simulink model "inv_psm"  (R2026b)
settings: Solver=ode23tb  StopTime=param.sim.simlength  FixedStep=param.sim.tc  MaxStep=param.glb_time.tc
values from neighbouring files (symbols this model uses):
  param = struct()    [init_model.m]
undefined symbols (not defined in the file or in its folder): magnitude
libraries: fl_lib x155, nesl_utility x77, igbt_simple_2th_lib x6, lithium_ion_battery x2, simple_flexible_shaft x2, cstblocks_lti x2, dclink_with_center_tap x1, three_phase_pwm_modulator x1, three_phase_inverter_ideal_switch_based_model x1, three_phase_inverter_igbt_advanced_thermal_model x1, three_phase_inverter_mosfet_based_with_thermal_model x1, threephase_inductor_lib x1
(part 6 of 6)

== system inv_psm/inv_psm_mod1/inverter_ctrl/inverter_control/current_ctrl/current_ctrl/dq_pi_with_vector_antiwindup mod1/dq_vector_pi/vector lenght ==
  md : Inport
  mq : Inport  Port=2
  Math Function : Math  Operator=magnitude^2  SignedPower=on
  Math Function1 : Math  Operator=magnitude^2  SignedPower=on
  Math Function2 : Math  Operator=reciprocal  SignedPower=on
  Sqrt : Sqrt
  Sum5 : Sum  SaturateOnIntegerOverflow=on
  m_1 : Outport  VectorParamsAs1DForOutWhenUnconnected=off
  m : Outport  Port=2  VectorParamsAs1DForOutWhenUnconnected=off
  wires:
  Sqrt/1 -> m/1, Math Function2/1
  mq/1 -> Math Function1/1
  Math Function1/1 -> Sum5/2
  Math Function/1 -> Sum5/1
  Sum5/1 -> Sqrt/1
  Math Function2/1 -> m_1/1
  md/1 -> Math Function/1

== system inv_psm/inv_psm_mod1/inverter_ctrl/inverter_control/current_ctrl/current_ctrl/dq_pi_with_vector_antiwindup mod1/dq_vector_pi_ccaller/Reset ==
  Step : Step  Time=0.05  InitialValue=1  FinalValue=0
  en : Outport
  wires:
  Step/1 -> en/1

== system inv_psm/inv_psm_mod1/inverter_ctrl/inverter_control/current_ctrl/bemf_observer/EKF_bemf_observer/extended_kalman_observer/correlation_matrix/A_ekf ==
  Gain1 : Gain  Gain=param.psm.ctrl.ekf.A6_tilde_ekf
  Gain{7..10,13,20} (6 alike) : Gain  Gain=param.psm.machine.omega_bez
  Gain{2,4,6,11,16,18} (6 alike) : Gain  Gain=param.glb_time.ts_inv
  Gain15 : Gain  Gain=param.psm.ctrl.ekf.A2_tilde_ekf
  Gain17 : Gain  Gain=param.psm.ctrl.ekf.A3_tilde_ekf
  Gain3 : Gain  Gain=param.psm.ctrl.ekf.A4_tilde_ekf
  Gain5 : Gain  Gain=param.psm.ctrl.ekf.A5_tilde_ekf
  I1 : Constant  Value=eye(6)
  I2 : Constant  Value=param.psm.ctrl.ekf.A1_tilde_ekf
  Sum7 : Sum  Inputs=+++++++
  out : Outport
  wires:
  Sum7/1 -> out/1
  I2/1 -> Gain11/1
  I1/1 -> Sum7/1
  Gain1/1 -> Gain2/1
  Gain3/1 -> Gain4/1
  Gain5/1 -> Gain6/1
  [omega_hat_kalman] -> Gain1/1
  [psi_alpha_hat] -> Gain3/1
  [psi_beta_hat] -> Gain5/1
  Gain11/1 -> Gain7/1
  Gain2/1 -> Gain8/1
  Gain4/1 -> Gain9/1
  Gain6/1 -> Gain10/1
  Gain7/1 -> Sum7/2
  Gain9/1 -> Sum7/5
  Gain10/1 -> Sum7/6
  Gain8/1 -> Sum7/7
  Gain18/1 -> Gain13/1
  Gain16/1 -> Gain20/1
  Gain17/1 -> Gain18/1
  Gain15/1 -> Gain16/1
  Gain13/1 -> Sum7/4
  Gain20/1 -> Sum7/3
  [i_beta_hat] -> Gain17/1
  [i_alpha_hat] -> Gain15/1

== matlab function inv_psm/inv_psm_mod1/inverter_ctrl/inverter_control/encoder-sensorless-switch/MATLAB Function ==
  data: omega_ctrl output; phase_psm input; omega_obs input; phase_obs input; phase_ctrl output; omega_psm input; omega_th input
function [omega_ctrl, phase_ctrl] = switch_enc2obs(phase_psm, omega_obs, phase_obs, omega_psm, omega_th)

if abs(omega_psm) > omega_th
    omega_ctrl = omega_obs;
    phase_ctrl = phase_obs;
else
    omega_ctrl = omega_psm;
    phase_ctrl = phase_psm;
end

== matlab function inv_psm/inv_psm_mod1/inverter_ctrl/inverter_control/encoder-sensorless-switch/double_integrator_observer/bounder1 ==
  data: u input; y output
function y = bounder(u)
    y = -pi + mod(u+3*pi,2*pi);
end

== matlab function inv_psm/inv_psm_mod1/inverter_ctrl/inverter_control/encoder-sensorless-switch/double_integrator_observer/bounder2 ==
  data: u input; y output
function y = bounder(u)
    y = -pi + mod(u+3*pi,2*pi);
end

== matlab function inv_psm/inv_psm_mod1/inverter_ctrl/inverter_control/current_ctrl/bemf_observer/EKF_bemf_observer/extended_kalman_observer/double_integrator_observer/bounder1 ==
  data: u input; y output
function y = bounder(u)
    y = -pi + mod(u+3*pi,2*pi);
end

== matlab function inv_psm/inv_psm_mod1/inverter_ctrl/inverter_control/current_ctrl/current_transformation/alphabeta2dq ==
  data: alpha input; d output; beta input; gamma input; q output
function [d,q] = alphabeta2dq(alpha,beta,gamma)

    d  =  alpha*cos(gamma) + beta*sin(gamma);
    q = -alpha*sin(gamma) + beta*cos(gamma);

end

== matlab function inv_psm/inv_psm_mod1/inverter_ctrl/inverter_control/current_ctrl/current_transformation/uvw2alphabeta ==
  data: u input; alpha output; v input; w input; beta output
function [alpha,beta] = uvw2alphabeta(u,v,w)

alpha = 2/3*(u - 1/2*v - 1/2*w);
beta  = 2/3*(sqrt(3)/2*(v - w));

end

== matlab function inv_psm/inv_psm_mod1/inverter_ctrl/inverter_control/current_ctrl/current_ctrl/output voltage transformation/dq2alphabeta ==
  data: d input; alpha output; q input; gamma input; beta output
function [alpha,beta] = dq2alphabeta(d,q,gamma)

    alpha  =  d*cos(gamma) - q*sin(gamma);
    beta = d*sin(gamma) + q*cos(gamma);

end

== matlab function inv_psm/inv_psm_mod1/inverter_ctrl/inverter_control/current_ctrl/bemf_observer/EKF_bemf_observer/extended_kalman_observer/double_integrator_observer/bounder2 ==
  data: u input; y output
function y = bounder(u)
    y = -pi + mod(u+3*pi,2*pi);
end

== matlab function inv_psm/inv_psm_mod1/inverter_ctrl/inverter_control/current_ctrl/bemf_observer/bemf_observer/double_integrator_observer/bounder1 ==
  data: u input; y output
function y = bounder(u)
    
    y = -pi + mod(u+3*pi,2*pi);
end

== matlab function inv_psm/inv_psm_mod1/inverter_ctrl/inverter_control/current_ctrl/bemf_observer/bemf_observer/double_integrator_observer/bounder2 ==
  data: u input; y output
function y = bounder(u)
    
    u = -pi + mod(u+3*pi,2*pi);
    
    y = u;
end
